simulink model "BatteryManagementSystem_MIL_TestModel"  (R2024a)
settings: Solver=VariableStepAuto  StartTime=0.0  StopTime=3600*4  RelTol=1e-3
InitFcn:
  | Capacity = 2.65;
  | c_rate= 0.5;
  | Np = 1; % Number of parallel cells
  | Ns = 3; % Number of series cells
  | voltageMin= 3.2;
  | currentThreshold = Capacity*Np/30;
  | voltageThreshold = 4.3;
  | CV_gain = 1;
  | voltageTolerance = 2;
undefined symbols (not defined in the file or in its folder): DiscIntNeverNeededParam, SRE
libraries: fl_lib x5, nesl_utility x5, Batteries_lib x1
settings Model: Creator=MANSY  LastModifiedBy=MANSY
settings OptimizationCC: DefaultUnderspecifiedDataType=single

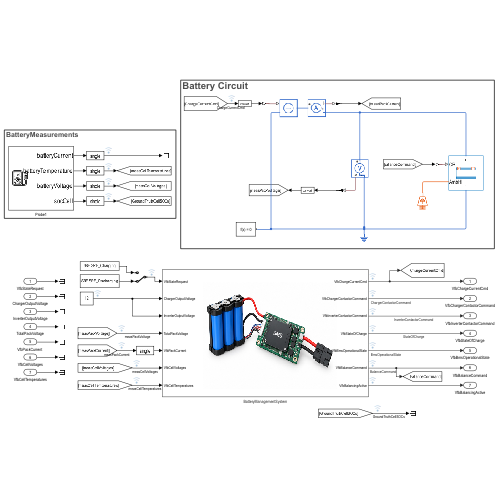
[thumbnail: Simulink's stored preview of the top-level diagram]
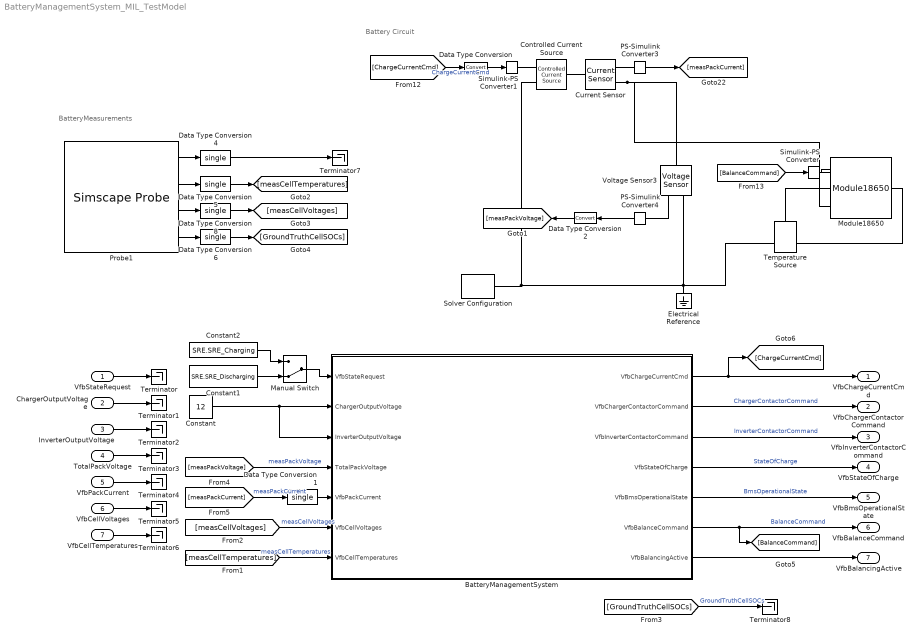
== system BatteryManagementSystem_MIL_TestModel ==
  note: Battery Circuit
  note: BatteryMeasurements
  VfbStateRequest : Inport
  ChargerOutputVoltage : Inport  Port=2
  InverterOutputVoltage : Inport  Port=3
  TotalPackVoltage : Inport  Port=4
  "VfbPackCurrent " : Inport  Port=5
  VfbCellVoltages : Inport  Port=6
  VfbCellTemperatures : Inport  Port=7
  BatteryManagementSystem : Subsystem
      mask Display: image('Lithium-Ion Battery BMS Module.png');
  Constant : Constant  Value=12  OutDataTypeStr=single
  Constant1 : Constant  Value=SRE.SRE_Discharging  OutDataTypeStr=Enum: SRE
  Constant2 : Constant  Value=SRE.SRE_Charging  OutDataTypeStr=Enum: SRE
  Controlled Current Source : fl_lib/Electrical/Electrical Sources/Controlled Current Source
  Current Sensor : fl_lib/Electrical/Electrical Sensors/Current Sensor
  Data Type Conversion : DataTypeConversion  SaturateOnIntegerOverflow=off  RndMeth=Floor
  Data Type Conversion{1,4..6,8} (5 alike) : DataTypeConversion  OutDataTypeStr=single  SaturateOnIntegerOverflow=off  RndMeth=Floor
  Data Type Conversion2 : DataTypeConversion  SaturateOnIntegerOverflow=off  RndMeth=Floor
  Electrical Reference : fl_lib/Electrical/Electrical Elements/Electrical Reference
  Manual Switch : ManualSwitch  CurrentSetting=0
  Module18650 : Batteries_lib/Module18650  BatteryCapacityCell=2.65 A*hr  ExtrapolationMethodCell=simscape.enum.extrapolation.linear  SOCBreakpointsCell=[0, .01, .02, .03, .04, .05, .06, .07, .08, .09, .1, .11, .12, .13, .14, .15, .16, .17, .18, .19, .2, .21, .22, .23, .24, .25, .26, .27, .28, .29, .3, .31, .32, .33, .34, .35, .36, .37, .38, .39, .4, .41, .42, .43, .44, .45, .46, .47, .48, .49, .5, .51, .52, .53, .54, .55, .56, .57, .58, .59, .6, .61, .62, .63, .64, .65, .66, .67, .68, .69, .7, .71, .72, .73, .74, .75, .76, .77, .78, .79, .8, .81, .82, .83, .84, .85, .86, .87, .88, .89, .9, .91, .92, .93, .94, .95, .96, .97, .98, .99, 1]  TemperatureBreakpointsCell=[0, 25, 40, 60] degC  OpenCircuitVoltageThermalCell=[3.04339, 3.04339, 3.04339, 3.04339; 3.19969, 3.19969, 3.19969, 3.19969; 3.32733, 3.32733, 3.32733, 3.32733; 3.41897, 3.41897, 3.41897, 3.41897; 3.47789, 3.47789, 3.47789, 3.47789; 3.5189, 3.5189, 3.5189, 3.5189; 3.54757, 3.54757, 3.54757, 3.54757; 3.56926, 3.56926, 3.56926, 3.56926; 3.58543, 3.58543, 3.58543, 3.58543; 3.59715, 3.59715, 3.59715, 3.59715; 3.60656, 3.60656, 3.60656, 3.60656; 3.61458, 3.61458, 3.61458, 3.61458; 3.62125, 3.62125, 3.62125, 3.62125; 3.62859, 3.62859, 3.62859, 3.62859; 3.63585, 3.63585, 3.63585, 3.63585; 3.64117, 3.64117, 3.64117, 3.64117; 3.64677, 3.64677, 3.64677, 3.64677; 3.65281, 3.65281, 3.65281, 3.65281; 3.65754, 3.65754, 3.65754, 3.65754; 3.6622, 3.6622, 3.6622, 3.6622; 3.66686, 3.66686, 3.66686, 3.66686; 3.67118, 3.67118, 3.67118, 3.67118; 3.67547, 3.67547, 3.67547, 3.67547; 3.67953, 3.67953, 3.67953, 3.67953; 3.68333, 3.68333, 3.68333, 3.68333; 3.68679, 3.68679, 3.68679, 3.68679; 3.68929, 3.68929, 3.68929, 3.68929; 3.69163, 3.69163, 3.69163, 3.69163; 3.69398, 3.69398, 3.69398, 3.69398; 3.69633, 3.69633, 3.69633, 3.69633; 3.69868, 3.69868, 3.69868, 3.69868; 3.70108, 3.70108, 3.70108, 3.70108; 3.7035, 3.7035, 3.7035, 3.7035; 3.70592, 3.70592, 3.70592, 3.70592; 3.70834, 3.70834, 3.70834, 3.70834; 3.71076, 3.71076, 3.71076, 3.71076; 3.71334, 3.71334, 3.71334, 3.71334; 3.71599, 3.71599, 3.71599, 3.71599; 3.71889, 3.71889, 3.71889, 3.71889; 3.72198, 3.72198, 3.72198, 3.72198; 3.72508, 3.72508, 3.72508, 3.72508; 3.72817, 3.72817, 3.72817, 3.72817; 3.73126, 3.73126, 3.73126, 3.73126; 3.73436, 3.73436, 3.73436, 3.73436; 3.73745, 3.73745, 3.73745, 3.73745; 3.74054, 3.74054, 3.74054, 3.74054; 3.74364, 3.74364, 3.74364, 3.74364; 3.74686, 3.74686, 3.74686, 3.74686; 3.75011, 3.75011, 3.75011, 3.75011; 3.75346, 3.75346, 3.75346, 3.75346; 3.75768, 3.75768, 3.75768, 3.75768; 3.7621, 3.7621, 3.7621, 3.7621; 3.76652, 3.76652, 3.76652, 3.76652; 3.77094, 3.77094, 3.77094, 3.77094; 3.77575, 3.77575, 3.77575, 3.77575; 3.78058, 3.78058, 3.78058, 3.78058; 3.78546, 3.78546, 3.78546, 3.78546; 3.79147, 3.79147, 3.79147, 3.79147; 3.79777, 3.79777, 3.79777, 3.79777; 3.80409, 3.80409, 3.80409, 3.80409; 3.8104, 3.8104, 3.8104, 3.8104; 3.81672, 3.81672, 3.81672, 3.81672; 3.82303, 3.82303, 3.82303, 3.82303; 3.82935, 3.82935, 3.82935, 3.82935; 3.83618, 3.83618, 3.83618, 3.83618; 3.84344, 3.84344, 3.84344, 3.84344; 3.8508, 3.8508, 3.8508, 3.8508; 3.85816, 3.85816, 3.85816, 3.85816; 3.86553, 3.86553, 3.86553, 3.86553; 3.87289, 3.87289, 3.87289, 3.87289; 3.88052, 3.88052, 3.88052, 3.88052; 3.88833, 3.88833, 3.88833, 3.88833; 3.89603, 3.89603, 3.89603, 3.89603; 3.90423, 3.90423, 3.90423, 3.90423; 3.91256, 3.91256, 3.91256, 3.91256; 3.92124, 3.92124, 3.92124, 3.92124; 3.93029, 3.93029, 3.93029, 3.93029; 3.93933, 3.93933, 3.93933, 3.93933; 3.94837, 3.94837, 3.94837, 3.94837; 3.95788, 3.95788, 3.95788, 3.95788; 3.96788, 3.96788, 3.96788, 3.96788; 3.97854, 3.97854, 3.97854, 3.97854; 3.98931, 3.98931, 3.98931, 3.98931; 4.00008, 4.00008, 4.00008, 4.00008; 4.01149, 4.01149, 4.01149, 4.01149; 4.02304, 4.02304, 4.02304, 4.02304; 4.03459, 4.03459, 4.03459, 4.03459; 4.04614, 4.04614, 4.04614, 4.04614; 4.05768, 4.05768, 4.05768, 4.05768; 4.06947, 4.06947, 4.06947, 4.06947; 4.08184, 4.08184, 4.08184, 4.08184; 4.09422, 4.09422, 4.09422, 4.09422; 4.1067, 4.1067, 4.1067, 4.1067; 4.11982, 4.11982, 4.11982, 4.11982; 4.1326, 4.1326, 4.1326, 4.1326; 4.14615, 4.14615, 4.14615, 4.14615; 4.15754, 4.15754, 4.15754, 4.15754; 4.16699, 4.16699, 4.16699, 4.16699; 4.17222, 4.17222, 4.17222, 4.17222; 4.18119, 4.18119, 4.18119, 4.18119; 4.30838, 4.30838, 4.30838, 4.30838] V  VoltageRangeCell=[2.7, Inf] V  ResistanceSOCBreakpointsCell=[0, .01, .02, .03, .04, .05, .06, .07, .08, .09, .1, .11, .12, .13, .14, .15, .16, .17, .18, .19, .2, .21, .22, .23, .24, .25, .26, .27, .28, .29, .3, .31, .32, .33, .34, .35, .36, .37, .38, .39, .4, .41, .42, .43, .44, .45, .46, .47, .48, .49, .5, .51, .52, .53, .54, .55, .56, .57, .58, .59, .6, .61, .62, .63, .64, .65, .66, .67, .68, .69, .7, .71, .72, .73, .74, .75, .76, .77, .78, .79, .8, .81, .82, .83, .84, .85, .86, .87, .88, .89, .9, .91, .92, .93, .94, .95, .96, .97, .98, .99, 1]  ResistanceTemperatureBreakpointsCell=[0, 25, 40, 60] degC  R0ThermalCell=[.10009, .04577, .01007, .01632; .14613, .0693, .01231, .013; .1823, .0871, .02576, .02712; .20605, .0981, .03749, .03657; .21852, .10274, .04624, .03593; .22481, .10473, .05239, .04275; .22685, .1047, .05724, .04532; .22648, .10401, .05969, .04893; .22421, .1029, .06023, .05216; .2204, .10084, .06022, .05386; .2158, .09855, .06061, .05477; .21072, .0961, .06053, .05519; .20518, .09374, .05997, .05515; .19986, .0923, .05976, .05534; .19452, .09098, .06051, .05551; .19005, .08942, .06059, .055; .18649, .08829, .06076, .05491; .18308, .08779, .06108, .05531; .17921, .08711, .06095, .05525; .17533, .08642, .06116, .05516; .17188, .08573, .06162, .05537; .16959, .08504, .06197, .05562; .16728, .08435, .0623, .05586; .16489, .08362, .06255, .05603; .16242, .08285, .06272, .0561; .15982, .0821, .06284, .05605; .15726, .08136, .06262, .05568; .15524, .08067, .06235, .05525; .15322, .07998, .06208, .05483; .1512, .07929, .06181, .05441; .14918, .07859, .06154, .05399; .14718, .07791, .06129, .05359; .14518, .07723, .06105, .05316; .14319, .07655, .06062, .05273; .14155, .07588, .06014, .0523; .14028, .0752, .05965, .05186; .13906, .07463, .05921, .05149; .13787, .07414, .0588, .05114; .13676, .07372, .05848, .05087; .13572, .07333, .05823, .05067; .13469, .07295, .05797, .05047; .13365, .07256, .05771, .05028; .13261, .07218, .05746, .0497; .13157, .07179, .0572, .04908; .13053, .07141, .05667, .04845; .12949, .07102, .05603, .04793; .1286, .07064, .05539, .04744; .12808, .07034, .05479, .04699; .12757, .07007, .0542, .04656; .1271, .06981, .05364, .04615; .12693, .06973, .05339, .04605; .12682, .0697, .0532, .04601; .12672, .06966, .05301, .04589; .12661, .06963, .05283, .04564; .12664, .06966, .05277, .04553; .12668, .06969, .05273, .04542; .12673, .06974, .0527, .04507; .12716, .07, .05306, .04491; .12758, .07016, .053, .04485; .128, .07032, .0529, .04479; .12841, .07047, .0528, .04474; .12883, .07062, .0527, .04468; .12925, .07078, .05261, .04463; .12967, .07093, .05251, .04457; .13027, .07117, .05259, .04469; .13101, .0715, .05282, .04497; .13204, .07186, .05308, .04484; .13321, .07221, .05335, .04472; .13439, .07256, .0532, .04459; .13557, .07292, .05301, .04446; .13684, .07332, .05292, .04443; .13817, .07375, .05288, .04428; .13946, .0741, .05281, .04407; .14091, .07448, .05291, .04404; .14233, .07489, .05306, .04405; .14388, .07535, .05333, .04418; .14556, .07584, .05372, .04444; .14723, .07633, .05411, .0447; .14891, .07682, .0545, .04496; .15108, .07759, .05506, .04537; .15372, .07866, .05578, .04596; .15659, .07988, .05673, .04678; .1595, .08112, .0574, .04703; .16241, .08236, .05796, .04728; .16616, .08368, .05874, .04774; .17134, .08499, .05957, .04825; .17651, .0863, .0604, .04877; .18169, .08761, .06123, .04928; .18774, .08891, .06206, .04979; .19646, .09039, .06297, .05038; .20538, .09225, .06408, .05118; .2143, .09411, .0652, .05198; .22836, .09597, .06593, .05281; .24309, .09796, .06644, .05348; .25899, .0995, .06683, .05394; .28056, .10104, .06749, .05466; .30009, .10043, .0674, .05464; .31508, .09826, .06607, .05332; .32861, .09216, .06054, .05002; .31916, .08512, .05631, .04686; .33322, .00997, .09284, .03396] Ohm  BatteryThermalMassCell=44.1 J/K  AmbientResistance=25 K/W  CellBalancingClosedResistance=0.01 Ohm  CellBalancingOpenConductance=1e-8 1/Ohm  CellBalancingThreshold=0.5  CellBalancingResistance=10 Ohm  P=1  S=3  SeriesGrouping=[1, 1, 1]  ParallelGrouping=[1, 1, 1]  socCell_specify=on  socCell_priority=High  socCell=[0.1 0.12 0.15]  socCell_nominal_specify=off  socCell_nominal_value=1  socCell_nominal_unit=1  numCycles_specify=off  numCycles_priority=High  numCycles=repmat(0, 3, 1)  numCycles_nominal_specify=off  numCycles_nominal_value=1  numCycles_nominal_unit=1  batteryVoltage_specify=off  batteryVoltage_priority=None  batteryVoltage=repmat(0, 3, 1) V  batteryVoltage_nominal_specify=off  batteryVoltage_nominal_value=1  batteryVoltage_nominal_unit=V  batteryCurrent_specify=off  batteryCurrent_priority=None  batteryCurrent=repmat(0, 3, 1) A  batteryCurrent_nominal_specify=off  batteryCurrent_nominal_value=1  batteryCurrent_nominal_unit=A  batteryTemperature_specify=off  batteryTemperature_priority=High  batteryTemperature=repmat(298.15, 3, 1) K  batteryTemperature_nominal_specify=off  batteryTemperature_nominal_value=1  batteryTemperature_nominal_unit=K  vParallelAssembly_specify=off  vParallelAssembly_priority=None  vParallelAssembly=repmat(0, 3, 1) V  vParallelAssembly_nominal_specify=off  vParallelAssembly_nominal_value=1  vParallelAssembly_nominal_unit=V  socParallelAssembly_specify=off  socParallelAssembly_priority=None  socParallelAssembly=repmat(1, 3, 1)  socParallelAssembly_nominal_specify=off  socParallelAssembly_nominal_value=1  socParallelAssembly_nominal_unit=1
      settings: InternalSimscapePortConfiguration="{\"Bottom\":[{\"id\":\"n\",\"label\":\"-\",\"type\":\"foundation.electrical.electrical\"}],\"Left\":[{\"id\":\"enableCellBalancing\",\"label\":\"CB\",\"type\":\"input\"},{\"id\":\"AmbH\",\"label\":\"AmbH\",\"type\":\"foundation.thermal.thermal\"}],\"Right\":[],\"Top\":[{\"id\":\"p\",\"label\":\"+\",\"type\":\"foundation.electrical.electrical\"}]}"
  PS-Simulink Converter3 : nesl_utility/PS-Simulink Converter  PhysicalDomain=network_engine_domain  SubClassName=ps_output  LeftPortType=input  RightPortType=output  PseudoPeriodic=off  Frequencies=[]  VectorFormat=inherit  Unit=inherit  AffineConversion=off
  PS-Simulink Converter4 : nesl_utility/PS-Simulink Converter  PhysicalDomain=network_engine_domain  SubClassName=ps_output  LeftPortType=input  RightPortType=output  PseudoPeriodic=off  Frequencies=[]  VectorFormat=inherit  Unit=inherit  AffineConversion=off
  Probe1 : SimscapeProbe  BoundBlock=738  Variables={batteryCurrent, batteryTemperature, batteryVoltage, socCell}
  Simulink-PS Converter : nesl_utility/Simulink-PS Converter  PhysicalDomain=network_engine_domain  SubClassName=ps_input  LeftPortType=input  RightPortType=output  PseudoPeriodic=off  Frequencies=[]  NoiseDistribution=none  NoiseParameters=[]  Unit=1  AffineConversion=off  FilteringAndDerivatives=provide  SimscapeFilterOrder=1  InputFilterTimeConstant=0.001  UdotUserProvided=0
  Simulink-PS Converter1 : nesl_utility/Simulink-PS Converter  PhysicalDomain=network_engine_domain  SubClassName=ps_input  LeftPortType=input  RightPortType=output  PseudoPeriodic=off  Frequencies=[]  NoiseDistribution=none  NoiseParameters=[]  Unit=1  AffineConversion=off  FilteringAndDerivatives=provide  SimscapeFilterOrder=1  InputFilterTimeConstant=0.001  UdotUserProvided=0
  Solver Configuration : nesl_utility/Solver Configuration  PhysicalDomain=network_engine_domain  SubClassName=solver  LeftPortType=input  RightPortType=generic  Tones=[]  Harmonics=[]  SimulateNoise=off  Profile=off  UseLocalSampling=off  EnableSwitchedLinearOptims=on  FrequencyDomain=off  UseCCode=off  RelTol=0.001  AbsTol=0.001  MinStep=1e-09  ToWorkspace=off  RevertToSquareIcSolve=off  NumHomotopyIterations=100  PhasorMode=off  PhasorModeNumHarmonics=1  ConsistencySolver=NEWTON_XTOL_AFTER_FTOL  IndexReductionMethod=DerivativeReplacement  DoDC=off  ResidualTolerance=1e-09  ConsistencyTolSource=GLOBAL  ConsistencyAbsTol=0.001  ConsistencyRelTol=0.001  ConsistencyTolFactor=0.001  UseLocalSolver=off  LocalSolverChoice=NE_BACKWARD_EULER_ADVANCER  ResolveIndetEquations=on  FunctionEvalNumThread=1  LocalSolverSampleTime=0.001  DoFixedCost=off  MaxNonlinIter=3  MaxModeIter=2  ComputeImpulses=off  ImpulseIterations=2  LinearAlgebra=auto  LinearAlgebraNumThread=0  EquationFormulation=NE_TIME_EF  DelaysMemoryBudget=1024  AutomaticFiltering=on  FilteringTimeConstant=0.001  PartitionStorageMethod=AS_NEEDED  PartitionMemoryBudget=1024  PartitionMethod=ROBUST  MultibodyUseLocalSolver=off  MultibodyLocalSolverChoice=ODE1  MultibodyLocalSolverSampleTime=0.001
  Temperature Source : fl_lib/Thermal/Thermal Sources/Temperature Source  temperature=30 degC
  Terminator{,1..8} (9 alike) : Terminator
  Voltage Sensor3 : fl_lib/Electrical/Electrical Sensors/Voltage Sensor
  VfbChargeCurrentCmd : Outport  OutDataTypeStr=single
  VfbChargerContactorCommand : Outport  Port=2  OutDataTypeStr=boolean
  VfbInverterContactorCommand : Outport  Port=3  OutDataTypeStr=boolean
  VfbStateOfCharge : Outport  Port=4  OutDataTypeStr=single
  VfbBmsOperationalState : Outport  Port=5
  VfbBalanceCommand : Outport  Port=6
  VfbBalancingActive : Outport  Port=7
  wires:
  [BalanceCommand] -> Simulink-PS Converter/1
  [ChargeCurrentCmd] -> Data Type Conversion/1  "ChargeCurrentCmd"
  Data Type Conversion5/1 -> [measCellTemperatures]
  Probe1/1 -> Data Type Conversion4/1
  Data Type Conversion8/1 -> [measCellVoltages]
  Data Type Conversion4/1 -> Terminator7/1
  Probe1/4 -> Data Type Conversion6/1
  Data Type Conversion6/1 -> [GroundTruthCellSOCs]
  PS-Simulink Converter3/1 -> [measPackCurrent]
  Probe1/2 -> Data Type Conversion5/1
  Probe1/3 -> Data Type Conversion8/1
  PS-Simulink Converter4/1 -> Data Type Conversion2/1
  VfbStateRequest/1 -> Terminator/1
  ChargerOutputVoltage/1 -> Terminator1/1
  InverterOutputVoltage/1 -> Terminator2/1
  TotalPackVoltage/1 -> Terminator3/1
  "VfbPackCurrent "/1 -> Terminator4/1
  VfbCellVoltages/1 -> Terminator5/1
  VfbCellTemperatures/1 -> Terminator6/1
  [measCellTemperatures] -> BatteryManagementSystem/7(VfbCellTemperatures)  "measCellTemperatures"
  [measCellVoltages] -> BatteryManagementSystem/6(VfbCellVoltages)  "measCellVoltages"
  [measPackVoltage] -> BatteryManagementSystem/4(TotalPackVoltage)  "measPackVoltage"
  Constant/1 -> BatteryManagementSystem/3(InverterOutputVoltage), BatteryManagementSystem/2(ChargerOutputVoltage)
  BatteryManagementSystem/6(VfbBalanceCommand) -> VfbBalanceCommand/1, [BalanceCommand]  "BalanceCommand"
  BatteryManagementSystem/1(VfbChargeCurrentCmd) -> [ChargeCurrentCmd], VfbChargeCurrentCmd/1
  BatteryManagementSystem/2(VfbChargerContactorCommand) -> VfbChargerContactorCommand/1  "ChargerContactorCommand"
  BatteryManagementSystem/3(VfbInverterContactorCommand) -> VfbInverterContactorCommand/1  "InverterContactorCommand"
  BatteryManagementSystem/4(VfbStateOfCharge) -> VfbStateOfCharge/1  "StateOfCharge"
  BatteryManagementSystem/5(VfbBmsOperationalState) -> VfbBmsOperationalState/1  "BmsOperationalState"
  BatteryManagementSystem/7(VfbBalancingActive) -> VfbBalancingActive/1
  [GroundTruthCellSOCs] -> Terminator8/1  "GroundTruthCellSOCs"
  Data Type Conversion/1 -> Simulink-PS Converter1/1
  [measPackCurrent] -> Data Type Conversion1/1  "measPackCurrent"
  Data Type Conversion1/1 -> BatteryManagementSystem/5("VfbPackCurrent ")
  Data Type Conversion2/1 -> [measPackVoltage]
  Manual Switch/1 -> BatteryManagementSystem/1(VfbStateRequest)
  Constant1/1 -> Manual Switch/2
  Constant2/1 -> Manual Switch/1
  connections:
  Solver Configuration/RConn1 -- Electrical Reference/LConn1 -- Voltage Sensor3/RConn2 -- Module18650/RConn1 -- Controlled Current Source/RConn2
  Current Sensor/RConn2 -- Module18650/LConn3 -- Voltage Sensor3/LConn1
  PS-Simulink Converter4/LConn1 -- Voltage Sensor3/RConn1
  Temperature Source/LConn1 -- Module18650/LConn2
  PS-Simulink Converter3/LConn1 -- Current Sensor/RConn1
  Simulink-PS Converter/RConn1 -- Module18650/LConn1
  Controlled Current Source/LConn1 -- Current Sensor/LConn1
  Simulink-PS Converter1/RConn1 -- Controlled Current Source/RConn1

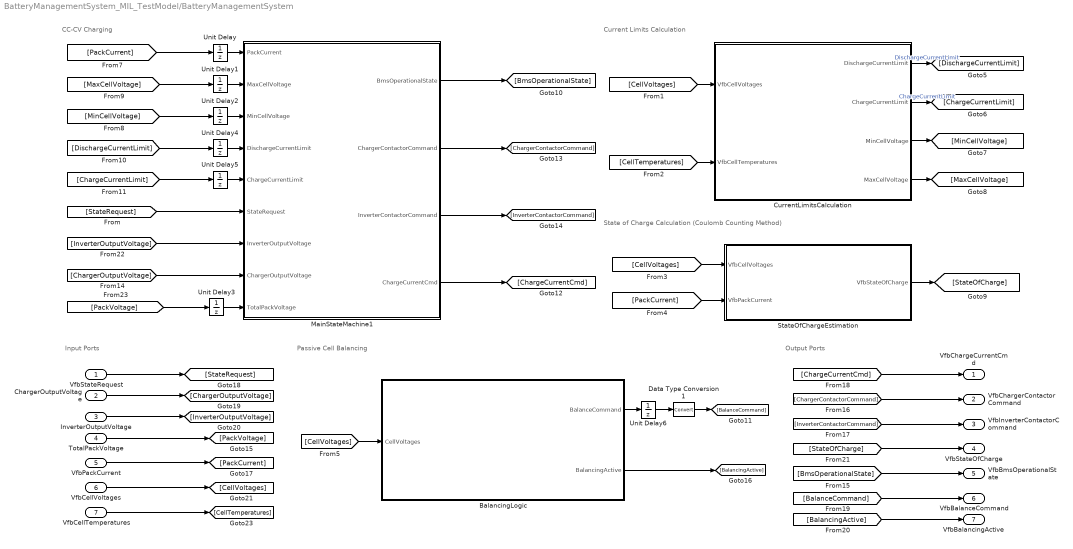
== system BatteryManagementSystem_MIL_TestModel/BatteryManagementSystem ==
  note: Passive Cell Balancing
  note: State of Charge Calculation (Coulomb Counting Method)
  note: Current Limits Calculation
  note: CC-CV Charging
  note: Output Ports
  note: Input Ports
  VfbStateRequest : Inport
  ChargerOutputVoltage : Inport  Port=2
  InverterOutputVoltage : Inport  Port=3
  TotalPackVoltage : Inport  Port=4
  "VfbPackCurrent " : Inport  Port=5
  VfbCellVoltages : Inport  Port=6
  VfbCellTemperatures : Inport  Port=7
  " StateOfChargeEstimation" : Subsystem  TreatAsAtomicUnit=on  SystemSampleTime=200e-3
      mask Display: image('SOC_img.png');
  BalancingLogic : MATLAB Function  TreatAsAtomicUnit=on  SystemSampleTime=250e-3
  "CurrentLimitsCalculation " : Subsystem  TreatAsAtomicUnit=on  SystemSampleTime=100e-3
      mask Display: image('CurrentLimit_img.png');
  Data Type Conversion1 : DataTypeConversion  SaturateOnIntegerOverflow=off  RndMeth=Floor
  MainStateMachine1 : Stateflow chart  TreatAsAtomicUnit=on  SystemSampleTime=50e-3
      settings: PortSchema="{\"entries\":[{\"content\":{\"sides\":[{\"content\":{\"connectorIds\":[\"In1\",\"In2\",\"In3\",\"In5\",\"In4\",\"In6\",\"In8\",\"In7\",\"In9\"]},\"type\":\"ConnectorPlacement.EquallySpacedRectSide\",\"uuid\":\"093f55e8-f90e-4d40-b8fb-904662301821\"},{\"content\":{\"connectorIds\":[\"Out1\",\"Out2\",\"Out3\",\"Out4\"],\"side\":\"RIGHT\"},\"type\":\"ConnectorPlacement.EquallySpacedRectSide\",\"uuid\":\"5101bd8f-b6b7-43f5-a647-8a1816a9003d\"},{\"content\":{\"side\":\"TOP\"},\"type\":\"ConnectorPlacement.EquallySpacedRectSide\",\"uuid\":\"c14aa96a-7f57-47da-866c-602a285b1131\"}]},\"type\":\"ConnectorPlacement.EquallySpacedConnector\",\"uuid\":\"8109f1a5-bcb4-40d5-94fc-489b7534b704\"}],\"packageUris\":[\"http://schema.mathworks.com/mf0/Connector/R2020b\"],\"version\":\"1.0\"}"
  Unit Delay{,1..6} (7 alike) : UnitDelay  SampleTime=-1  HasFrameUpgradeWarning=on
  VfbChargeCurrentCmd : Outport  OutDataTypeStr=single
  VfbChargerContactorCommand : Outport  Port=2  OutDataTypeStr=boolean
  VfbInverterContactorCommand : Outport  Port=3  OutDataTypeStr=boolean
  VfbStateOfCharge : Outport  Port=4  OutDataTypeStr=single
  VfbBmsOperationalState : Outport  Port=5
  VfbBalanceCommand : Outport  Port=6
  VfbBalancingActive : Outport  Port=7
  wires:
  TotalPackVoltage/1 -> [PackVoltage]
  MainStateMachine1/3(InverterContactorCommand) -> [InverterContactorCommand]
  [CellVoltages] -> "CurrentLimitsCalculation "/1(VfbCellVoltages)
  [BalancingActive] -> VfbBalancingActive/1
  "VfbPackCurrent "/1 -> [PackCurrent]
  "CurrentLimitsCalculation "/4(MaxCellVoltage) -> [MaxCellVoltage]
  [StateOfCharge] -> VfbStateOfCharge/1
  [InverterContactorCommand] -> VfbInverterContactorCommand/1
  [PackCurrent] -> Unit Delay/1
  MainStateMachine1/4(ChargeCurrentCmd) -> [ChargeCurrentCmd]
  Unit Delay5/1 -> MainStateMachine1/4(ChargeCurrentLimit)
  Data Type Conversion1/1 -> [BalanceCommand]
  [BalanceCommand] -> VfbBalanceCommand/1
  [ChargerContactorCommand] -> VfbChargerContactorCommand/1
  [InverterOutputVoltage] -> MainStateMachine1/8(InverterOutputVoltage)
  Unit Delay3/1 -> MainStateMachine1/9(TotalPackVoltage)
  [BmsOperationalState] -> VfbBmsOperationalState/1
  [StateRequest] -> MainStateMachine1/6(StateRequest)
  BalancingLogic/1(BalanceCommand) -> Unit Delay6/1
  BalancingLogic/2(BalancingActive) -> [BalancingActive]
  [DischargeCurrentLimit] -> Unit Delay4/1
  [ChargeCurrentCmd] -> VfbChargeCurrentCmd/1
  [ChargerOutputVoltage] -> MainStateMachine1/7(ChargerOutputVoltage)
  [ChargeCurrentLimit] -> Unit Delay5/1
  Unit Delay/1 -> MainStateMachine1/1(PackCurrent)
  Unit Delay1/1 -> MainStateMachine1/2(MaxCellVoltage)
  [CellTemperatures] -> "CurrentLimitsCalculation "/2(VfbCellTemperatures)
  [PackCurrent] -> " StateOfChargeEstimation"/2("VfbPackCurrent ")
  InverterOutputVoltage/1 -> [InverterOutputVoltage]
  Unit Delay6/1 -> Data Type Conversion1/1
  MainStateMachine1/2(ChargerContactorCommand) -> [ChargerContactorCommand]
  [MaxCellVoltage] -> Unit Delay1/1
  VfbCellVoltages/1 -> [CellVoltages]
  [PackVoltage] -> Unit Delay3/1
  VfbCellTemperatures/1 -> [CellTemperatures]
  [CellVoltages] -> BalancingLogic/1(CellVoltages)
  [CellVoltages] -> " StateOfChargeEstimation"/1(VfbCellVoltages)
  MainStateMachine1/1(BmsOperationalState) -> [BmsOperationalState]
  [MinCellVoltage] -> Unit Delay2/1
  "CurrentLimitsCalculation "/2(ChargeCurrentLimit) -> [ChargeCurrentLimit]  "ChargeCurrentLimit"
  ChargerOutputVoltage/1 -> [ChargerOutputVoltage]
  "CurrentLimitsCalculation "/1(DischargeCurrentLimit) -> [DischargeCurrentLimit]  "DischargeCurrentLimit"
  " StateOfChargeEstimation"/1(VfbStateOfCharge) -> [StateOfCharge]
  Unit Delay4/1 -> MainStateMachine1/5(DischargeCurrentLimit)
  VfbStateRequest/1 -> [StateRequest]
  Unit Delay2/1 -> MainStateMachine1/3(MinCellVoltage)
  "CurrentLimitsCalculation "/3(MinCellVoltage) -> [MinCellVoltage]

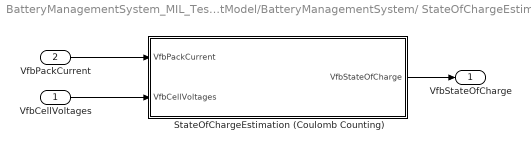
== system BatteryManagementSystem_MIL_TestModel/BatteryManagementSystem/ StateOfChargeEstimation ==
  VfbCellVoltages : Inport
  "VfbPackCurrent " : Inport  Port=2
  StateOfChargeEstimation (Coulomb Counting) : Subsystem  TreatAsAtomicUnit=on
  VfbStateOfCharge : Outport
  wires:
  StateOfChargeEstimation (Coulomb Counting)/1(VfbStateOfCharge) -> VfbStateOfCharge/1
  "VfbPackCurrent "/1 -> StateOfChargeEstimation (Coulomb Counting)/1("VfbPackCurrent ")
  VfbCellVoltages/1 -> StateOfChargeEstimation (Coulomb Counting)/2(VfbCellVoltages)

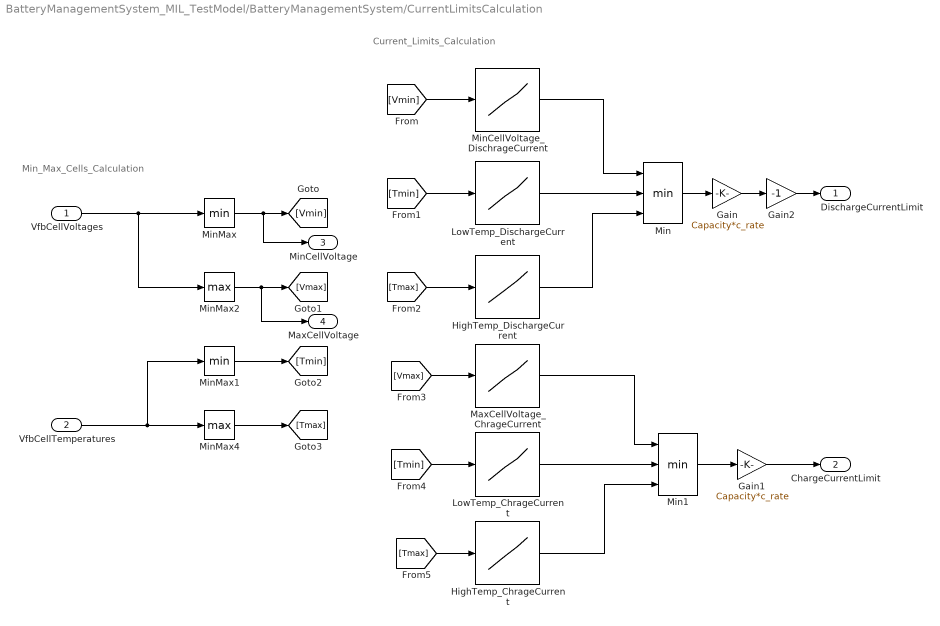
== system BatteryManagementSystem_MIL_TestModel/BatteryManagementSystem/CurrentLimitsCalculation  ==
  note: Current_Limits_Calculation
  note: Min_Max_Cells_Calculation
  VfbCellVoltages : Inport  OutDataTypeStr=single  PortDimensions=3
  VfbCellTemperatures : Inport  Port=2  OutDataTypeStr=single  PortDimensions=3
  Gain : Gain  Gain=Capacity*c_rate
  Gain1 : Gain  Gain=Capacity*c_rate
  Gain2 : Gain  Gain=-1
  HighTemp_ChrageCurrent : Lookup_n-D  NumberOfTableDimensions=1  BreakpointsForDimension1=single([298.15 308.15 313.15 318.15 323.15 333.15])  Table=single([1 1 0.8 0.5 0.2 0])  InternalRulePriority=Speed  RndMeth=Simplest
  HighTemp_DischargeCurrent : Lookup_n-D  NumberOfTableDimensions=1  BreakpointsForDimension1=single([298.15 308.15 313.15 318.15 323.15 333.15])  Table=single([1 1 0.9 0.7 0.4 0])  InternalRulePriority=Speed  RndMeth=Simplest
  LowTemp_ChrageCurrent : Lookup_n-D  NumberOfTableDimensions=1  BreakpointsForDimension1=single([243.15 263.15 273.15 278.15 283.15 288.15 298.15])  Table=single([0 0 0 0.1 0.3 0.6 1])  InternalRulePriority=Speed  RndMeth=Simplest
  LowTemp_DischargeCurrent : Lookup_n-D  NumberOfTableDimensions=1  BreakpointsForDimension1=single([243.15 258.15 273.15 283.15 293.15 298.15])  Table=single([0 0 0.2 0.6 0.9 1])  InternalRulePriority=Speed  RndMeth=Simplest
  MaxCellVoltage_ChrageCurrent : Lookup_n-D  NumberOfTableDimensions=1  BreakpointsForDimension1=single([3.0 3.5 3.8 4.0 4.1 4.2 4.25 4.35])  Table=single([1 1 1 0.9 0.7 0.4 0.2 0])  InternalRulePriority=Speed  RndMeth=Simplest
  Min : MinMax  Inputs=3
  Min1 : MinMax  Inputs=3
  MinCellVoltage_DischrageCurrent : Lookup_n-D  NumberOfTableDimensions=1  BreakpointsForDimension1=single([2.7 2.8 3.0 3.2 3.4 3.6])  Table=single([0 0.1 0.3 0.6 0.9 1])  InternalRulePriority=Speed  RndMeth=Simplest
  MinMax : MinMax
  MinMax1 : MinMax
  MinMax2 : MinMax  Function=max
  MinMax4 : MinMax  Function=max
  DischargeCurrentLimit : Outport  OutDataTypeStr=single
  ChargeCurrentLimit : Outport  Port=2  OutDataTypeStr=single
  MinCellVoltage : Outport  Port=3
  MaxCellVoltage : Outport  Port=4
  wires:
  [Vmin] -> MinCellVoltage_DischrageCurrent/1
  Gain/1 -> Gain2/1
  VfbCellVoltages/1 -> MinMax2/1, MinMax/1
  LowTemp_ChrageCurrent/1 -> Min1/2
  [Tmin] -> LowTemp_ChrageCurrent/1
  MinMax4/1 -> [Tmax]
  [Tmin] -> LowTemp_DischargeCurrent/1
  [Tmax] -> HighTemp_ChrageCurrent/1
  Min1/1 -> Gain1/1
  MaxCellVoltage_ChrageCurrent/1 -> Min1/1
  MinMax/1 -> MinCellVoltage/1, [Vmin]
  LowTemp_DischargeCurrent/1 -> Min/2
  MinMax2/1 -> MaxCellVoltage/1, [Vmax]
  HighTemp_DischargeCurrent/1 -> Min/3
  HighTemp_ChrageCurrent/1 -> Min1/3
  Gain1/1 -> ChargeCurrentLimit/1
  [Tmax] -> HighTemp_DischargeCurrent/1
  Min/1 -> Gain/1
  [Vmax] -> MaxCellVoltage_ChrageCurrent/1
  MinCellVoltage_DischrageCurrent/1 -> Min/1
  VfbCellTemperatures/1 -> MinMax4/1, MinMax1/1
  MinMax1/1 -> [Tmin]
  Gain2/1 -> DischargeCurrentLimit/1

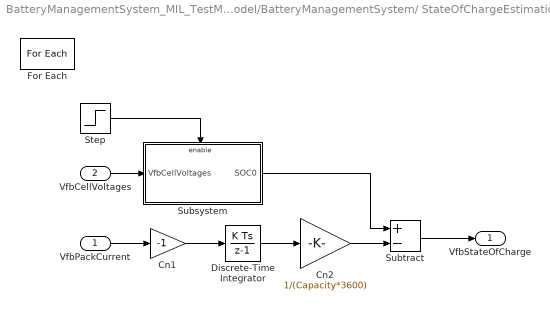
== system BatteryManagementSystem_MIL_TestModel/BatteryManagementSystem/ StateOfChargeEstimation/StateOfChargeEstimation (Coulomb Counting) ==
  "VfbPackCurrent " : Inport  OutDataTypeStr=single
  VfbCellVoltages : Inport  Port=2  Partition=on  PartitionDimension=1  PartitionWidth=1  PartitionOffset=0
  Cn1 : Gain  Gain=-1  OutDataTypeStr=single
  Cn2 : Gain  Gain=1/(Capacity*3600)  OutDataTypeStr=single
  Discrete-Time Integrator : DiscreteIntegrator  gainval=1  SampleTime=-1  OutDataTypeStr=single  RndMeth=Nearest  ICPrevOutput=DiscIntNeverNeededParam  ICPrevScaledInput=DiscIntNeverNeededParam
  For Each : ForEach  DisableCoverage=on
  Step : Step  Time=0.1  Before=1  After=0
  Subsystem : Subsystem
  Subtract : Sum  Inputs=+-
  VfbStateOfCharge : Outport  OutDataTypeStr=single  ConcatenationDimension=1
  wires:
  Cn1/1 -> Discrete-Time Integrator/1
  Discrete-Time Integrator/1 -> Cn2/1
  "VfbPackCurrent "/1 -> Cn1/1
  Subtract/1 -> VfbStateOfCharge/1
  Subsystem/1(SOC0) -> Subtract/1
  Step/1 -> Subsystem/Enable
  VfbCellVoltages/1 -> Subsystem/1(VfbCellVoltages)
  Cn2/1 -> Subtract/2

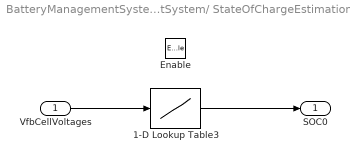
== system BatteryManagementSystem_MIL_TestModel/BatteryManagementSystem/ StateOfChargeEstimation/StateOfChargeEstimation (Coulomb Counting)/Subsystem ==
  VfbCellVoltages : Inport
  Enable : EnablePort
  1-D Lookup Table3 : Lookup_n-D  NumberOfTableDimensions=1  BreakpointsForDimension1=|  Table=|  InternalRulePriority=Speed  RndMeth=Simplest
      BreakpointsForDimension1=|
      | [3.04339, 3.19969, 3.32733, 3.41897, 3.47789, 3.5189, ...
      | 3.54757, 3.56926, 3.58543, 3.59715, 3.60656, 3.61458, ...
      | 3.62125, 3.62859, 3.63585, 3.64117, 3.64677, 3.65281, ...
      | 3.65754, 3.6622, 3.66686, 3.67118, 3.67547, 3.67953, ...
      | 3.68333, 3.68679, 3.68929, 3.69163, 3.69398, 3.69633, ...
      | 3.69868, 3.70108, 3.7035, 3.70592, 3.70834, 3.71076, ...
      | 3.71334, 3.71599, 3.71889, 3.72198, 3.72508, 3.72817, ...
      | 3.73126, 3.73436, 3.73745, 3.74054, 3.74364, 3.74686, ...
      | 3.75011, 3.75346, 3.75768, 3.7621, 3.76652, 3.77094, ...
      | 3.77575, 3.78058, 3.78546, 3.79147, 3.79777, 3.80409, ...
      | 3.8104, 3.81672, 3.82303, 3.82935, 3.83618, 3.84344, ...
      | 3.8508, 3.85816, 3.86553, 3.87289, 3.88052, 3.88833, ...
      | 3.89603, 3.90423, 3.91256, 3.92124, 3.93029, 3.93933, ...
      | 3.94837, 3.95788, 3.96788, 3.97854, 3.98931, 4.00008, ...
      | 4.01149, 4.02304, 4.03459, 4.04614, 4.05768, 4.06947, ...
      | 4.08184, 4.09422, 4.1067, 4.11982, 4.1326, 4.14615, ...
      | 4.15754, 4.16699, 4.17222, 4.18119, 4.30838]
      Table=|
      | [0, 0.01, 0.02, 0.03, 0.04, 0.05, 0.06, 0.07, 0.08, 0.09, ...
      | 0.10, 0.11, 0.12, 0.13, 0.14, 0.15, 0.16, 0.17, 0.18, 0.19, ...
      | 0.20, 0.21, 0.22, 0.23, 0.24, 0.25, 0.26, 0.27, 0.28, 0.29, ...
      | 0.30, 0.31, 0.32, 0.33, 0.34, 0.35, 0.36, 0.37, 0.38, 0.39, ...
      | 0.40, 0.41, 0.42, 0.43, 0.44, 0.45, 0.46, 0.47, 0.48, 0.49, ...
      | 0.50, 0.51, 0.52, 0.53, 0.54, 0.55, 0.56, 0.57, 0.58, 0.59, ...
      | 0.60, 0.61, 0.62, 0.63, 0.64, 0.65, 0.66, 0.67, 0.68, 0.69, ...
      | 0.70, 0.71, 0.72, 0.73, 0.74, 0.75, 0.76, 0.77, 0.78, 0.79, ...
      | 0.80, 0.81, 0.82, 0.83, 0.84, 0.85, 0.86, 0.87, 0.88, 0.89, ...
      | 0.90, 0.91, 0.92, 0.93, 0.94, 0.95, 0.96, 0.97, 0.98, 0.99, 1]
  SOC0 : Outport
  wires:
  VfbCellVoltages/1 -> 1-D Lookup Table3/1
  1-D Lookup Table3/1 -> SOC0/1

== stateflow chart BatteryManagementSystem_MIL_TestModel/BatteryManagementSystem/MainStateMachine1 ==
  state Charging
    entry:
    BmsOperationalState = BMS_State_Enum.Charging;
    ChargerContactorCommand =1;
    exit:
    ChargerContactorCommand =0;
    state CC
      entry:
      ChargeCurrentCmd = ChargeCurrentLimit;
    state CV
      during:
      ChargeCurrentCmd = ChargeCurrentCmd - CV_gain*(MaxCellVoltage - voltageThreshold);
      ChargeCurrentCmd = min(ChargeCurrentCmd, ChargeCurrentLimit);
    (default) -> CC
    CC -> CV : [MaxCellVoltage > voltageThreshold]
  state Discharging
    entry:
    InverterContactorCommand = 1;
    BmsOperationalState = BMS_State_Enum.Discharging;
    during:
    ChargeCurrentCmd = DischargeCurrentLimit;
    exit:
    InverterContactorCommand = 0;
  state Standby
    entry:
    ChargeCurrentCmd = 0;
    BmsOperationalState = BMS_State_Enum.Standby;
    InverterContactorCommand =0;
    ChargerContactorCommand =0;
  Discharging -> Charging [order 1] : [StateRequest ==	SRE.SRE_Charging && abs(ChargerOutputVoltage - TotalPackVoltage) < voltageTolerance]
  Charging -> Discharging [order 2] : [StateRequest ==	SRE.SRE_Discharging && abs(InverterOutputVoltage - TotalPackVoltage ) < voltageTolerance && abs(ChargerOutputVoltage - TotalPackVoltage) < voltageTolerance]
  Standby -> Discharging [order 1] : [(StateRequest ==	SRE.SRE_Discharging) && (MinCellVoltage > 1.1*voltageMin) && (abs(InverterOutputVoltage - TotalPackVoltage ) < voltageTolerance) ]
  Discharging -> Standby [order 2] : [ StateRequest ==	SRE.SRE_Standby || MinCellVoltage < voltageMin ]
  (default) -> Standby
  Charging -> Standby [order 1] : [ StateRequest ==	SRE.SRE_Standby || PackCurrent < currentThreshold ]
  Standby -> Charging [order 2] : [StateRequest ==	SRE.SRE_Charging && MinCellVoltage < 0.95*voltageThreshold && abs(ChargerOutputVoltage - TotalPackVoltage) < voltageTolerance]
  data: CV_gain parameter single; currentThreshold parameter single; voltageMin parameter single; voltageThreshold parameter single; PackCurrent input single; MaxCellVoltage input single; MinCellVoltage input single; ChargeCurrentLimit input single; DischargeCurrentLimit input single; StateRequest input Enum: SRE; BmsOperationalState output Enum: BMS_State_Enum; voltageTolerance parameter single; ChargerOutputVoltage input single; InverterOutputVoltage input single; TotalPackVoltage input single; ChargerContactorCommand output boolean; InverterContactorCommand output boolean; ChargeCurrentCmd output single

== matlab function BatteryManagementSystem_MIL_TestModel/BatteryManagementSystem/BalancingLogic ==
  data: CellVoltages input; BalanceCommand output boolean; BalancingActive output
function [BalanceCommand,BalancingActive]= fcn(CellVoltages)
Vmin = min(CellVoltages);
BalanceCommand = false(size(CellVoltages));
BalancingActive = false;
deltaV_threshold = 0.05;
for i = 1: length(CellVoltages)
   deltaV = CellVoltages(i)-Vmin;
   BalanceCommand(i) = deltaV >deltaV_threshold;
end

BalancingActive = any(BalanceCommand);

end
